simulink model "TempControl_closed_loop"  (R2026b)
settings: Solver=FixedStepDiscrete  StopTime=250  FixedStep=10e-3  EnableMultiTasking=on
values from neighbouring files (symbols this model uses):
  Ki_zn = Kp_zn / Tn_zn    [prep_lab_2.m]
  Kp_zn = 0.9 * tau / (K * Tt_zn)    [prep_lab_2.m]
libraries: mbedblockslib x2, cstblocks_lti x1, slpidlib x1
settings Model: SILPILModeSetting=veronly  Creator=Lukas  LastModifiedBy=ursmu
settings OptimizationCC: DifferentSizesBufferReuse=on  EnhancedBackFolding=on  MaxStackSize=64  OptimizationCustomize=off  OptimizeBlockOrder=speed
settings DebuggingCC: ParameterTunabilityLossMsg=error
settings HardwareCC: ProdHWDeviceType=ARM Compatible->ARM Cortex  ProdLargestAtomicFloat=Double  ProdLargestAtomicInteger=Long  ProdLongLongMode=on
settings SFSimCC: MATLABDynamicMemAlloc=off
settings RTWCC: Description=Embedded Coder  HardwareBoard=STM32 Nucleo F401RE  SystemTargetFile=ert.tlc  TLCOptions=-aInlineSetEventsForThisBaseRateFcn=TLC_FALSE -aSuppressMultiTaskScheduler=TLC_FALSE -aRateBasedStepFcn=1  TemplateMakefile=ert_default_tmf  Toolchain=GNU Tools for STM32
settings CodeAppCC: ForceParamTrailComments=on  OperatorAnnotations=on
settings ERTTargetCC: CodeReplacementLibrary=ARM Cortex-M  DynamicArrayContainerType=coder::array  ERTCustomFileBanners=off  ExtModeIntrfLevel=Level2 - Open  ExtModeMexFile=ext_xcp  ExtModeStaticAlloc=on  ModelStepFunctionPrototypeControlCompliant=off  SupportContinuousTime=on  SupportNonInlinedSFcns=on

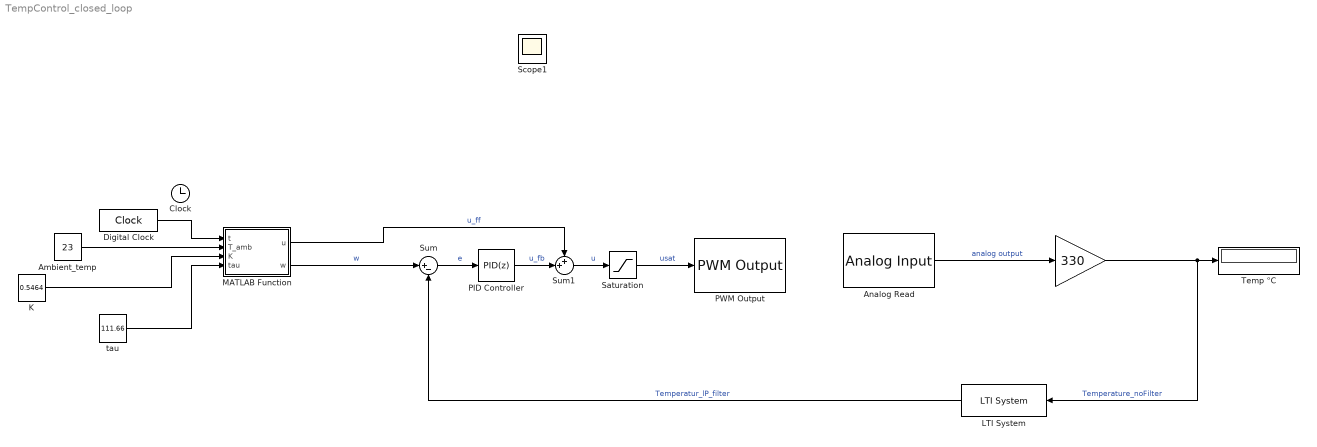
== system TempControl_closed_loop ==
  " " : Gain  Gain=330
  Ambient_temp : Constant  Value=23
  Analog Read : mbedblockslib/Analog Input  Pin=A0  ReadResultsOnly=off  ConversionTriggerSource=Software  ExternalTriggerType=uint32( 0 )  OutputDataType=double  EnableConversionCompleteNotify=off  EnableOuputStatus=off  SampleTime=10e-3
      settings: LibrarySourceBlock=stmnucleorootlib/Common/Analog Input
  Clock : Clock
  Digital Clock : DigitalClock  SampleTime=0.01
  K : Constant  Value=0.5464
  LTI System : cstblocks_lti/LTI System  sys=lowpass_z  IC=[]  PadeOrder=0
      settings: LibrarySourceBlock=cstblocks/Linear Time Invariant/LTI System
  MATLAB Function : MATLAB Function  TreatAsAtomicUnit=on
  PID Controller : slpidlib/PID Controller  Controller=PID  Form=Parallel  TimeDomain=Discrete-time  UseExternalTs=off  SampleTime=-1  IntegratorMethod=Forward Euler  FilterMethod=Forward Euler  ControllerParametersSource=internal  P=Kp_zn  I=Ki_zn  UseKiTs=off  D=0  UseExternalDerivativeSource=off  N=100  UseFilter=on  TunerSelectOption=Transfer Function Based (PID Tuner App)  InitialConditionSource=internal  InitialConditionForIntegrator=0  InitialConditionForFilter=0  DifferentiatorICPrevScaledInput=0  ExternalReset=none  TrackingMode=off  Kt=1  LimitOutput=off  SatLimitsSource=internal  UpperSaturationLimit=inf  LowerSaturationLimit=-inf  LinearizeAsGain=on  AntiWindupMode=none  Kb=1  LimitIntegrator=off  UpperIntegratorSaturationLimit=inf  LowerIntegratorSaturationLimit=-inf  POutMin=[]  POutMax=[]  IOutMin=[]  IOutMax=[]  DOutMin=[]  DOutMax=[]  NOutMin=[]  NOutMax=[]  SumOutMin=[]  SumOutMax=[]  SaturationOutMin=[]  SaturationOutMax=[]  PParamMin=[]  PParamMax=[]  IParamMin=[]  IParamMax=[]  DParamMin=[]  DParamMax=[]  NParamMin=[]  NParamMax=[]  KbParamMin=[]  KbParamMax=[]  KtParamMin=[]  KtParamMax=[]  KbOutMin=[]  KbOutMax=[]  KtOutMin=[]  KtOutMax=[]  IntegratorOutMin=[]  IntegratorOutMax=[]  FilterOutMin=[]  FilterOutMax=[]  SumI1OutMin=[]  SumI1OutMax=[]  SumI2OutMin=[]  SumI2OutMax=[]  SumI3OutMin=[]  SumI3OutMax=[]  SumI4OutMin=[]  SumI4OutMax=[]  SumDOutMin=[]  SumDOutMax=[]  DifferentiatorOutMin=[]  DifferentiatorOutMax=[]  FilterDiffOutCoefMin=[]  FilterDiffOutCoefMax=[]  ReciprocalOutMin=[]  ReciprocalOutMax=[]  SumDenOutMin=[]  SumDenOutMax=[]  SumNumOutMin=[]  SumNumOutMax=[]  DivideOutMin=[]  DivideOutMax=[]  UdiffTsProdOutMin=[]  UdiffTsProdOutMax=[]  NTsProdOutMin=[]  NTsProdOutMax=[]  UintegralTsProdOutMin=[]  UintegralTsProdOutMax=[]  UngainTsProdOutMin=[]  UngainTsProdOutMax=[]  ClampingZeroOutDataTypeStr=Inherit: Inherit via back propagation  ClampingZeroOutMin=[]  ClampingZeroOutMax=[]  FilterDenConstantOutDataTypeStr=Inherit: Inherit via back propagation  FilterDenConstantOutMin=[]  FilterDenConstantOutMax=[]  PCopyOutDataTypeStr=Inherit: Inherit via back propagation  PCopyOutMin=[]  PCopyOutMax=[]  NCopyOutDataTypeStr=Inherit: Inherit via back propagation  NCopyOutMin=[]  NCopyOutMax=[]  IntegratorContinuousStateAttributes=''  IntegratorStateMustResolveToSignalObject=off  IntegratorRTWStateStorageClass=Auto  FilterContinuousStateAttributes=''  FilterStateMustResolveToSignalObject=off  FilterRTWStateStorageClass=Auto  ParallelPVariant=InternalParameters  IdealPVariant=Disabled  IVariant=InternalParameters  DVariant=InternalParameters  IntegratorVariant=Discrete  SatVariant=Disabled  AWVariant=Passthrough  PCopyVariant=Disabled  TRVariant=Disabled  FdbkBlocksVariant=Forward  IdealPFdbkVariant=Disabled  SatFdbkVariant=Disabled  DerivativeFilterVariant=ForwardEulerFilter  NVariant=InternalParameters  NCopyVariant=Disabled  FilterICVariant=InternalICsFilter  IntegratorICVariant=InternalICs  ExternalResetVariant=Disabled  TRSumVariant=Passthrough  SumFdbkVariant=Disabled  SumVariant=Sum_PID  TsampFilterVariant=InternalTs  TsampNgainVariant=Passthrough  TsampIntegralVariant=Disabled_SignalSpec  ExternalSaturationOutDataTypeStr=Inherit: Same as second input  DerivativeSourceVariant=ErrorSignal  PreIntVariant=InternalPreInt
  PWM Output : mbedblockslib/PWM Output  Pin=D2  EnableInputFrequency=off  InitialFrequency=10000  InitialDutyCycle=20  NotificationType=None
      settings: LibrarySourceBlock=stmnucleorootlib/Common/PWM Output
  Saturation : Saturate  UpperLimit=100  LowerLimit=0
  Sum : Sum  Inputs=|+-
  Sum1 : Sum  Inputs=++|
  Temp °C : Display
  tau : Constant  Value=111.66
  Scope1 : Scope
      settings: ActiveDisplayYMinimum=20.9423  ActiveDisplayYMaximum=22.6548
  wires:
  Analog Read/1 -> " "/1  "analog output"
  " "/1 -> LTI System/1, Temp °C/1  "Temperature_noFilter"
  Sum/1 -> PID Controller/1  "e"
  Saturation/1 -> PWM Output/1  "usat"
  Digital Clock/1 -> MATLAB Function/1(t)
  MATLAB Function/2(w) -> Sum/1  "w"
  PID Controller/1 -> Sum1/2  "u_fb"
  MATLAB Function/1(u) -> Sum1/1  "u_ff"
  Sum1/1 -> Saturation/1  "u"
  Ambient_temp/1 -> MATLAB Function/2(T_amb)
  K/1 -> MATLAB Function/3(K)
  tau/1 -> MATLAB Function/4(tau)
  LTI System/1 -> Sum/2  "Temperatur_lP_filter"

== matlab function TempControl_closed_loop/MATLAB Function ==
  data: u output; w output; t input; T_amb input; K input; tau input
function [u, w] = fcn(t, T_amb, K, tau)
if (t >= 0) && (t < 80)
    dy_ref = 15 / 80;
    y_ref  = dy_ref * t;
elseif (t >= 80) && (t < 120)
    dy_ref = 0;
    y_ref  = 15;
elseif (t >= 120) && (t <= 240)
    dy_ref = -15 / 120;
    y_ref  = 15 + dy_ref * (t - 120);
else
    dy_ref = 0;
    y_ref  = 0;
end
w = T_amb + y_ref;
u = (y_ref + tau * dy_ref) / K;
end
